simulink model "Maxom_fcs_noncascaded"  (R2025b)
settings: Solver=ode45  StartTime=0.0  StopTime=0.30  FixedStep=1e-6  MaxStep=1e-5  RelTol=1e-4  EnableMultiTasking=on
values from neighbouring files (symbols this model uses):
  Bfric = 0    [PMSMpara.m]
  ffai = 0.008667    [PMSMpara.m]
  Imax = 20    [PMSMpara.m]
  J = 0.044e-4    (= 4.4e-06)    [PMSMpara.m]
  kis = 0    [PMSMpara.m]
  kps = fsc*6.28*J/Kt    (= 0.364364007978)    [PMSMpara.m]
  Kt = np*1.5*ffai    (= 0.0910035)    [PMSMpara.m]
  Ld = Ls    (= 0.00045)    [PMSMpara.m]
  Lq = Ls    (= 0.00045)    [PMSMpara.m]
  np = 7    [PMSMpara.m]
  Rs = 0.5    [PMSMpara.m]
  Tcur = 1/32000    (= 3.125e-05)    [PMSMpara.m]
  Tpwm = 1/32000    (= 3.125e-05)    [PMSMpara.m]
  Tspd = 1/32000    (= 3.125e-05)    [PMSMpara.m]
  wn = 311040    [PMSMpara.m]
  zeta = 1    [PMSMpara.m]
undefined symbols (not defined in the file or in its folder): dspblkCoreblockFVToolHelper, gcbh
libraries: simulink x4, slpidlib x2, spsUniversalBridgeLib x1, spsCurrentMeasurementLib x1, EasyGo_Machine_lib x1, spsPermanentMagnetSynchronousMachineLib x1, spsSVPWMGenerator2LevelLib x1, spsDCVoltageSourceLib x1, sps_lib x1
(part 3 of 4)

== matlab function Maxom_fcs_noncascaded/f_pmsm_foc_sl/MATLAB Function12 ==
  data: ia input; gg output; ib input; ic input; id_ref input; we_ref input; we input; TL_hat input; theta_m input; Vdc input; Ld input; Lq input; Rs input; lambda_f input; Jm input; Bfric input; Tcur input; lambda_w input; lambda_id input; lambda_sw input; we_scale input; i_scale input; iq_max input; i_pred output; we_pred output; we_spread output
function [gg, i_pred, we_pred, we_spread] = fcs_noncascade_np3( ...
    ia, ib, ic, id_ref, we_ref, we, TL_hat, theta_m, ...
    Vdc, Ld, Lq, Rs, lambda_f, Jm, Bfric, Tcur, lambda_w,...
    lambda_id, lambda_sw, we_scale, i_scale, iq_max)
%#codegen
% Non-cascade FCS-MPC, Np=3, full 8^3 enumeration, normalized cost.
% NOMINAL model (electrical SMDO removed): current recursion keeps -Rs*i,
% no lumped current-disturbance compensation. TL_hat still feed-forwards load.

np = single(7);
ia=single(ia); ib=single(ib); ic=single(ic);
id_ref=single(id_ref); we_ref=single(we_ref); we=single(we); TL_hat=single(TL_hat);
Vdc=single(Vdc); Ld=single(Ld); Lq=single(Lq); Rs=single(Rs); lambda_f=single(lambda_f);
Jm=single(Jm); Bfric=single(Bfric); Ts=single(Tcur);
lambda_id=single(lambda_id); lambda_sw=single(lambda_sw);
we_scale=single(we_scale); i_scale=single(i_scale); iq_max=single(iq_max);

theta_e = single(mod(np*theta_m - pi/2, 2*pi));
inv_Ld=single(1)/Ld; inv_Lq=single(1)/Lq; inv_J=single(1)/Jm;
TsLd=Ts*inv_Ld; TsLq=Ts*inv_Lq;
ct=single(cos(theta_e)); st=single(sin(theta_e));

% --- hoisted constants ---
Kt     = single(1.5)*np*lambda_f;
aRd    = single(1) - TsLd*Rs;
aRq    = single(1) - TsLq*Rs;
TsKJ   = Ts*np*inv_J;
aW     = single(1) - Ts*Bfric*inv_J;
inv_ws=single(1)/we_scale; inv_is=single(1)/i_scale;
imax2 = iq_max*iq_max;
BIGPEN=single(1e5);
lsw3  = lambda_sw/single(3);

% Clarke/Park (measured)
i_alpha=(single(2)/3)*(ia-single(0.5)*ib-single(0.5)*ic);
i_beta =(single(2)/3)*(single(sqrt(3))/2)*(ib-ic);
is_d= ct*i_alpha+st*i_beta;
is_q=-st*i_alpha+ct*i_beta;

V=single([0 0 0;1 0 0;1 1 0;0 1 0;0 1 1;0 0 1;1 0 1;1 1 1]);
Kcl=(single(2)/3)*Vdc*single([1 -0.5 -0.5;0 single(sqrt(3))/2 -single(sqrt(3))/2]);

persistent s_prev
if isempty(s_prev)
    s_prev=zeros(3,1,'single');
end

% ===== nominal model: no disturbance bias =====
bd = single(0);   % was Ts*d_hat_d from SMDO
bq = single(0);   % was Ts*d_hat_q from SMDO

% ===== 8 dq voltages, and per-vector current INCREMENTS =====
Vab=Kcl*V';
Vdq=single([ct st;-st ct])*Vab;      % 2x8
dVd = TsLd*Vdq(1,:);                  % 1x8
dVq = TsLq*Vdq(2,:);

% ===== 8x8 switching table + sw0 from s_prev =====
SW = zeros(8,8,'single');
for a=1:8
    for b=1:8
        SW(a,b)=abs(V(b,1)-V(a,1))+abs(V(b,2)-V(a,2))+abs(V(b,3)-V(a,3));
    end
end
sw0=zeros(8,1,'single');
for n=1:8
    sw0(n)=abs(V(n,1)-s_prev(1))+abs(V(n,2)-s_prev(2))+abs(V(n,3)-s_prev(3));
end

% ===== horizon-3 tree search =====
g_best=single(1e30); n1_best=int32(1);
id_best=single(0); iq_best=single(0); we_best1=single(0);
we_min1=single(1e30); we_max1=single(-1e30);

for n1=1:8
    id1 = aRd*is_d + dVd(n1);
    iq1 = aRq*is_q + bq + dVq(n1);
    Te1 = Kt*iq1;
    we1 = aW*we + TsKJ*(Te1 - TL_hat);
    if we1<we_min1, we_min1=we1; end
    if we1>we_max1, we_max1=we1; end
    ew=(we_ref-we1)*inv_ws;
    ei=(id_ref-id1)*inv_is;
    c1 = ew*ew + lambda_id*(ei*ei) + lsw3*sw0(n1);
    if (id1*id1+iq1*iq1)>imax2, c1=c1+BIGPEN; end

    for n2=1:8
        id2 = aRd*id1 + bd + dVd(n2);
        iq2 = aRq*iq1 + bq + dVq(n2);
        Te2 = Kt*iq2;
        we2 = aW*we1 + TsKJ*(Te2 - TL_hat);
        ew=(we_ref-we2)*inv_ws; ei=(id_ref-id2)*inv_is;
        c12 = c1 + ew*ew + lambda_id*(ei*ei) + lsw3*SW(n1,n2);
        if (id2*id2+iq2*iq2)>imax2, c12=c12+BIGPEN; end

        for n3=1:8
            id3 = aRd*id2 + bd + dVd(n3);
            iq3 = aRq*iq2 + bq + dVq(n3);
            Te3 = Kt*iq3;
            we3 = aW*we2 + TsKJ*(Te3 - TL_hat);
            ew=(we_ref-we3)*inv_ws;
            ei=(id_ref-id3)*inv_is;
            Jc = c12 + lambda_w*(ew*ew) + lambda_id*(ei*ei) + lsw3*SW(n2,n3);
            if (id3*id3+iq3*iq3)>imax2, Jc=Jc+BIGPEN; end

            if Jc<g_best
                g_best=Jc; n1_best=int32(n1);
                id_best=id1; iq_best=iq1; we_best1=we1;
            end
        end
    end
end

s_prev=V(n1_best,:)';
Sa=s_prev(1); Sb=s_prev(2); Sc=s_prev(3);
gg=single([Sa;1-Sa;Sb;1-Sb;Sc;1-Sc]);
i_pred=single([id_best;iq_best]);
we_pred=single(we_best1);
we_spread=single(we_max1-we_min1);
end

== matlab function Maxom_fcs_noncascaded/f_pmsm_foc_sl/MATLAB Function13 ==
  data: ia input; gg output; ib input; ic input; id_ref input; we_ref input; we input; TL_hat input; theta_m input; Vdc input; Ld input; Lq input; Rs input; lambda_f input; Jm input; Bfric input; Tcur input; lambda_w input; lambda_id input; lambda_sw input; we_scale input; i_scale input; iq_max input
function gg = fcs_noncascade_np3_fast( ...
    ia, ib, ic, id_ref, we_ref, we, TL_hat, theta_m, ...
    Vdc, Ld, Lq, Rs, lambda_f, Jm, Bfric, Tcur, lambda_w, ...
    lambda_id, lambda_sw, we_scale, i_scale, iq_max)
%#codegen
%GPT optimized, 70 microseconds

% Optimized non-cascade FCS-MPC, Np = 3.
%
% Full 8^3 search is retained.
%
% Branch-and-bound assumes:
% lambda_w >= 0, lambda_id >= 0, lambda_sw >= 0.

%% Type conversion
ia        = single(ia);
ib        = single(ib);
ic        = single(ic);
id_ref    = single(id_ref);
we_ref    = single(we_ref);
we        = single(we);
TL_hat    = single(TL_hat);
theta_m   = single(theta_m);

Vdc       = single(Vdc);
Ld        = single(Ld);
Lq        = single(Lq);
Rs        = single(Rs);
lambda_f  = single(lambda_f);
Jm        = single(Jm);
Bfric     = single(Bfric);
Ts        = single(Tcur);

lambda_w  = single(lambda_w);
lambda_id = single(lambda_id);
lambda_sw = single(lambda_sw);
we_scale  = single(we_scale);
i_scale   = single(i_scale);
iq_max    = single(iq_max);

one = single(1);
np  = single(7);

%% Persistent constant lookup tables
persistent S SW alpha_pu beta_pu previous_index

if isempty(previous_index)

    % Switching-state order:
    % 1:000  2:100  3:110  4:010
    % 5:011  6:001  7:101  8:111
    S = single([ ...
        0 0 0;
        1 0 0;
        1 1 0;
        0 1 0;
        0 1 1;
        0 0 1;
        1 0 1;
        1 1 1]);

    % Hamming distance between switching states
    SW = single([ ...
        0 1 2 1 2 1 2 3;
        1 0 1 2 3 2 1 2;
        2 1 0 1 2 3 2 1;
        1 2 1 0 1 2 3 2;
        2 3 2 1 0 1 2 1;
        1 2 3 2 1 0 1 2;
        2 1 2 3 2 1 0 1;
        3 2 1 2 1 2 1 0]);

    % Normalized inverter voltage vectors:
    % v_alpha = Vdc*alpha_pu
    % v_beta  = Vdc*beta_pu
    alpha_pu = single([ ...
         0, ...
         0.6666666667, ...
         0.3333333333, ...
        -0.3333333333, ...
        -0.6666666667, ...
        -0.3333333333, ...
         0.3333333333, ...
         0]);

    beta_pu = single([ ...
         0, ...
         0, ...
         0.5773502692, ...
         0.5773502692, ...
         0, ...
        -0.5773502692, ...
        -0.5773502692, ...
         0]);

    % Initial switching state is 000
    previous_index = int32(1);
end

%% Electrical angle
theta_e = mod( ...
    np*theta_m - single(pi/2), ...
    single(2*pi));

ct = cos(theta_e);
st = sin(theta_e);

%% Clarke-Park transformation
two_thirds = single(0.6666666667);
half       = single(0.5);
sqrt3_half = single(0.8660254038);

i_alpha = two_thirds*(ia - half*ib - half*ic);
i_beta  = two_thirds*sqrt3_half*(ib - ic);

is_d =  ct*i_alpha + st*i_beta;
is_q = -st*i_alpha + ct*i_beta;

%% Hoisted model constants
TsLd = Ts/Ld;
TsLq = Ts/Lq;

aRd = one - TsLd*Rs;
aRq = one - TsLq*Rs;
aW  = one - Ts*Bfric/Jm;

Kt = single(1.5)*np*lambda_f;

% Original:
% we_next = aW*we + Ts*np/Jm*(Kt*iq - TL_hat)
%
% Combined form:
bIq = Ts*np*Kt/Jm;
dTL = Ts*np*TL_hat/Jm;

imax2 = iq_max*iq_max;

BIGPEN = single(1e5);

% Cost coefficients
kw12 = one/(we_scale*we_scale);
kw3  = lambda_w*kw12;
kid  = lambda_id/(i_scale*i_scale);
ksw  = lambda_sw/single(3);

%% dq voltage increments
kVd = TsLd*Vdc;
kVq = TsLq*Vdc;

dVd = zeros(1,8,'single');
dVq = zeros(1,8,'single');

for n = 1:8
    vd_pu =  ct*alpha_pu(n) + st*beta_pu(n);
    vq_pu = -st*alpha_pu(n) + ct*beta_pu(n);

    dVd(n) = kVd*vd_pu;
    dVq(n) = kVq*vq_pu;
end

%% Initial upper bound: repeat the previous state three times
p = previous_index;

id1 = aRd*is_d + dVd(p);
iq1 = aRq*is_q + dVq(p);
we1 = aW*we + bIq*iq1 - dTL;

ew = we_ref - we1;
ei = id_ref - id1;

g_best = kw12*ew*ew + kid*ei*ei;

if id1*id1 + iq1*iq1 > imax2
    g_best = g_best + BIGPEN;
end

id2 = aRd*id1 + dVd(p);
iq2 = aRq*iq1 + dVq(p);
we2 = aW*we1 + bIq*iq2 - dTL;

ew = we_ref - we2;
ei = id_ref - id2;

g_best = g_best + kw12*ew*ew + kid*ei*ei;

if id2*id2 + iq2*iq2 > imax2
    g_best = g_best + BIGPEN;
end

id3 = aRd*id2 + dVd(p);
iq3 = aRq*iq2 + dVq(p);
we3 = aW*we2 + bIq*iq3 - dTL;

ew = we_ref - we3;
ei = id_ref - id3;

g_best = g_best + kw3*ew*ew + kid*ei*ei;

if id3*id3 + iq3*iq3 > imax2
    g_best = g_best + BIGPEN;
end

n1_best = previous_index;

%% Horizon-three branch-and-bound search
for n1 = 1:8

    id1 = aRd*is_d + dVd(n1);
    iq1 = aRq*is_q + dVq(n1);
    we1 = aW*we + bIq*iq1 - dTL;

    ew = we_ref - we1;
    ei = id_ref - id1;

    c1 = kw12*ew*ew + kid*ei*ei ...
       + ksw*SW(previous_index,n1);

    if id1*id1 + iq1*iq1 > imax2
        c1 = c1 + BIGPEN;
    end

    % All remaining terms are nonnegative
    if c1 >= g_best
        continue;
    end

    for n2 = 1:8

        id2 = aRd*id1 + dVd(n2);
        iq2 = aRq*iq1 + dVq(n2);
        we2 = aW*we1 + bIq*iq2 - dTL;

        ew = we_ref - we2;
        ei = id_ref - id2;

        c12 = c1 ...
            + kw12*ew*ew ...
            + kid*ei*ei ...
            + ksw*SW(n1,n2);

        if id2*id2 + iq2*iq2 > imax2
            c12 = c12 + BIGPEN;
        end

        if c12 >= g_best
            continue;
        end

        for n3 = 1:8

            id3 = aRd*id2 + dVd(n3);
            iq3 = aRq*iq2 + dVq(n3);
            we3 = aW*we2 + bIq*iq3 - dTL;

            ew = we_ref - we3;
            ei = id_ref - id3;

            Jc = c12 ...
               + kw3*ew*ew ...
               + kid*ei*ei ...
               + ksw*SW(n2,n3);

            if id3*id3 + iq3*iq3 > imax2
                Jc = Jc + BIGPEN;
            end

            if Jc < g_best
                g_best  = Jc;
                n1_best = int32(n1);
            end
        end
    end
end

%% Apply first optimal switching state
previous_index = n1_best;

Sa = S(n1_best,1);
Sb = S(n1_best,2);
Sc = S(n1_best,3);

gg = [ ...
    Sa;
    one-Sa;
    Sb;
    one-Sb;
    Sc;
    one-Sc];

end

== matlab function Maxom_fcs_noncascaded/original ==
  data: ia input; gg output; ib input; ic input; id_ref input; iq_ref input; omega_mech input; theta_mech input; Vdc input; Ld input; Lq input; Rs input; lambda_f input; Tpwm input; lambda_w input; id1 output; id2 output; iq1 output; iq2 output
function [gg, id1, id2, iq1, iq2]  = fcs_mpc_2step(ia, ib, ic, id_ref, iq_ref, ...
                                      omega_mech, theta_mech, Vdc, ...
                                      Ld, Lq, Rs, lambda_f, Tpwm, lambda_w)
%#codegen
% =========================================================================
% TWO-STEP-DELAY FCS-MPC  --  compensating the one-sample compute delay
% -------------------------------------------------------------------------
% MEANING. On real hardware the vector chosen this tick cannot act during
%   [k,k+1): that interval was already committed last tick. So instead of
%   optimising from the measurement x(k), first roll the model forward one
%   step under the already-applied vector to get x(k+1), then choose the
%   vector for [k+1,k+2) by scoring the prediction x(k+2). The chosen vector
%   is stored and applied next cycle (via the actuation delay). This is the
%   classic Cortes et al. two-step scheme; horizon is otherwise 1.
% NEED. Without it, the controller assumes its choice takes effect
%   instantly. The real one-sample lag then shows up as extra current ripple
%   and, at high speed / high fundamental frequency, degraded stability --
%   the model and the plant are literally one step out of phase.
% WHEN TO USE. Any real deployment where prediction + optimisation consumes
%   a meaningful fraction of the tick (i.e. essentially always on an MCU),
%   or any simulation that models the actuation with a unit delay (z^-1) on
%   the output. In an idealised, instantaneous-actuation simulation it is
%   unnecessary. The same "predict one step first" idea composes with the
%   long-horizon and observer variants.
% =========================================================================

omega_r = omega_mech*7;
theta_e = mod(theta_mech*7-pi/2, 2*pi);

Ts = Tpwm;

% eight 2-level VSI switching states {Sa,Sb,Sc}
i_alpha = (2/3)*(ia - 0.5*ib - 0.5*ic);
i_beta = (2/3)*(sqrt(3)/2*(ib - ic));

% Park (align d with rotor flux)
is_d =  cos(theta_e)*i_alpha + sin(theta_e)*i_beta;
is_q = -sin(theta_e)*i_alpha + cos(theta_e)*i_beta;

V = single([0 0 0; 1 0 0; 1 1 0; 0 1 0; 0 1 1; 0 0 1; 1 0 1; 1 1 1]);
Kcl = (2/3)*Vdc*single([1 -0.5 -0.5; 0 sqrt(3)/2 -sqrt(3)/2]);

persistent s_now % vector applied during [k,k+1)
if isempty(s_now), s_now = zeros(3,1,'single'); end

% step 1: predict x(k+1) under the already-committed vector
Pk  = single([cos(theta_e) sin(theta_e); -sin(theta_e) cos(theta_e)]);
v0  = Pk * (Kcl * s_now);
id1 = is_d + Ts/Ld*(-Rs*is_d + omega_r*Lq*is_q + v0(1));
iq1 = is_q + Ts/Lq*(-Rs*is_q - omega_r*Ld*is_d - omega_r*lambda_f + v0(2));

% step 2: choose the vector for [k+1,k+2) at the advanced angle
th1 = theta_e + omega_r*Ts;
P1  = single([cos(th1) sin(th1); -sin(th1) cos(th1)]);
%P2  = single([cos(th2) sin(th2); -sin(th2) cos(th2)]);
g_best = single(inf);  idx = int32(1);
id2 = single(0);  iq2 = single(0); % declare outside the loop
for n = 1:8
    v_dq = P1 * (Kcl * V(n,:)');
    id2c = id1 + Ts/Ld*(-Rs*id1 + omega_r*Lq*iq1 + v_dq(1));
    iq2c = iq1 + Ts/Lq*(-Rs*iq1 - omega_r*Ld*id1 - omega_r*lambda_f + v_dq(2));
    g = (id_ref - id2c)^2 + lambda_w*(iq_ref - iq2c)^2;
    if g < g_best
        g_best = g;  idx = int32(n);
        id2 = id2c;  iq2 = iq2c; % keep the CHOSEN prediction
    end
end

s_new = V(idx,:)';
s_now = s_new; % becomes the committed vector next tick
Sa = s_new(1);  Sb = s_new(2);  Sc = s_new(3);
gg = single([Sa; 1-Sa; Sb; 1-Sb; Sc; 1-Sc]);
end

== matlab function Maxom_fcs_noncascaded/MATLAB Function1 ==
  data: speed_ref_cmd input; iq_feedforward output
function iq_feedforward = fcn_speed_feedforward( speed_ref_cmd)
    % ----------------- 系统硬参数定义 -----------------
    FS = single(32000);               % 控制频率 32kHz
    DT = single(1)/ FS;            % 采样周期 31.25us
    POLE_PAIRS = single(7);           % 极对数
    MAX_CURRENT_LIMIT = single(20); % 最大限流 20A (用于限制最大加速度)

    % ----------------- 电机软参数定义 (需要实测/辨识) -----------------
    % 1. J_total: 电机转子+负载的总转动惯量 (单位: kg·m^2)
    J_total = single(0.044e-4*2);        % 【需根据实际系统调整】
    % 2. Kt: 电机转矩常数 (单位: N·m/A)。通常 Kt ≈ 反电动势常数 Ke
    Kt = single(0.091003);                % 【需根据电机规格书调整】

    % ----------------- 持久化状态变量 -----------------
    persistent prev_ramped_speed ramped_speed
    if isempty(ramped_speed)
        prev_ramped_speed = single(0);
        ramped_speed = single(0);
    end

    persistent prev_iq_ff
if isempty(prev_iq_ff)
    prev_iq_ff = single(0);
end


    % ========================================================
    % 【第一步：速度轨迹规划（生成平滑斜坡）】
    % ========================================================
    % 理论最大加速度限制：a_max = (Kt * Max_Current) / J_total
    max_accel_rpm_s = (Kt * MAX_CURRENT_LIMIT) / J_total * 60.0 / (2 * pi);

    % 跟随目标速度（做斜坡上升/下降限制）
    if speed_ref_cmd > ramped_speed
        ramped_speed = ramped_speed + max_accel_rpm_s * DT; % 加速
        if ramped_speed > speed_ref_cmd
            ramped_speed = speed_ref_cmd;
        end
    elseif speed_ref_cmd < ramped_speed
        ramped_speed = ramped_speed - max_accel_rpm_s * DT; % 减速
        if ramped_speed < speed_ref_cmd
            ramped_speed = speed_ref_cmd;
        end
    end

    % ========================================================
    % 【第二步：计算加速度前馈】
    % ========================================================
    % 1. 计算速度差分（得到实际需要的加速度）
    delta_rpm = ramped_speed - prev_ramped_speed;
    accel_rpm_s = delta_rpm / DT; % RPM / s

    % 2. 将加速度转换为 电角速度 变化率 (rad/s^2)
    accel_rad_s2 = accel_rpm_s * (2 * pi / 60.0) * POLE_PAIRS;

    % 3. 计算所需的前馈 Iq 电流 (基于牛顿第二定律: T = J * a, T = Kt * Iq)
    iq_raw = (J_total * accel_rad_s2) / Kt;

    % --- 引入前馈斜率限制（替代低通滤波，0相位滞后） ---

% 设定前馈电流的最大变化率（单位：A/s）
% 根据电机电气时间常数，建议从 500 ~ 2000 A/s 开始往下调
MAX_FF_SLEW_RATE = single(50000); 
max_delta_per_loop = MAX_FF_SLEW_RATE * DT; % 每个控制周期允许的最大电流变化

diff = iq_raw - prev_iq_ff;
if diff > max_delta_per_loop
    diff = max_delta_per_loop;
elseif diff < -max_delta_per_loop
    diff = -max_delta_per_loop;
end

% 得到平滑后的前馈（方波的垂直边变成了斜坡边）
iq_feedforward = prev_iq_ff + diff;

% 最后统一做安全限幅
iq_feedforward = max(-MAX_CURRENT_LIMIT, min(MAX_CURRENT_LIMIT, iq_feedforward));
prev_iq_ff = iq_feedforward;

    % 4. 安全限幅（防止前馈计算出超出硬件能力的电流）
    if iq_feedforward > MAX_CURRENT_LIMIT
        iq_feedforward = MAX_CURRENT_LIMIT;
    elseif iq_feedforward < -MAX_CURRENT_LIMIT
        iq_feedforward = -MAX_CURRENT_LIMIT;
    end

    % 更新状态
    prev_ramped_speed = ramped_speed;
end

== matlab function Maxom_fcs_noncascaded/MATLAB Function3 ==
  data: spd_ref input; iq_total output; spd_act input; iq_ff input
function iq_total = fcn_PI_FF_AntiWindup(spd_ref, spd_act, iq_ff)
    % ------------ 系统硬参数定义 ------------
    FS = single(32000);
    DT = single(1)/FS;  % 采样周期 31.25us
    Kp = single(1.5);   % 比例系数（请根据您原来 PID 的参数修改）
    Ki = single(50.0);  % 积分系数（请根据您原来 PID 的参数修改）
    
    MAX_LIM = single(20);    % 上限幅 (跟您外部的 20A 保持一致)
    MIN_LIM = single(-20);   % 下限幅
    
    persistent integral
    if isempty(integral)
        integral = single(0);
    end
    
    % 1. 计算速度误差
    error = spd_ref - spd_act;
    
    % 2. 计算 PI 输出 + 前馈 的总和
    iq_total_raw = (Kp * error + integral) + iq_ff;
    
    % 3. 对总和进行外部限幅
    if iq_total_raw > MAX_LIM
        iq_total = MAX_LIM;
    elseif iq_total_raw < MIN_LIM
        iq_total = MIN_LIM;
    else
        iq_total = iq_total_raw;
    end
    
    % 4. 【核心】：感知外部限幅的真实抗饱和策略
    % 如果触发了限幅，且误差方向还试图让限幅更深，则冻结积分器！
    if (iq_total >= MAX_LIM && error > 0) || (iq_total <= MIN_LIM && error < 0)
        integral = integral; % 冻结积分
    else
        integral = integral + Ki * error * DT; % 正常累加积分
    end
end

== matlab function Maxom_fcs_noncascaded/f_pmsm_foc_sl/MATLAB Function7 ==
  data: ia input; gg output; ib input; ic input; id_ref input; iq_ref input; omega_mech input; theta_mech input; Vdc input; Ld input; Lq input; Rs input; lambda_f input; Tcur input; lambda_w input; Va output; Vb output; Vc output
function [gg, Va, Vb, Vc] = fcs_smdo_2step(ia, ib, ic, id_ref, iq_ref, ...
                                     omega_mech, theta_mech, Vdc, Ld, Lq, Rs, ...
                                     lambda_f, Tcur, lambda_w)
%#codegen
% ---- horizon & dims (INTEGERS — do not make these single) --------------
Np   = int32(3);            % prediction horizon
dim  = int32(3 * Np);
ny   = int32(2);
nyNp = int32(ny * Np);

% ---- pole pairs & electrical quantities (separate from horizon) --------
omega_r  = single(omega_mech*7);               % electrical if external np gain applied;
theta_e = mod(theta_mech*7 - pi/2, 2*pi);
Ts = single(Tcur);

% Clarke + Park
i_alpha = (2/3)*(ia - 0.5*ib - 0.5*ic);
i_beta  = (2/3)*(sqrt(3)/2*(ib - ic));
is_d =  cos(theta_e)*i_alpha + sin(theta_e)*i_beta;
is_q = -sin(theta_e)*i_alpha + cos(theta_e)*i_beta;


% ---- constants that were input ports in v2 -----------------------------
lambda_u = single(1e-3);     % switching-effort weight; 0 = pure tracking to start
en_pwm   = true;            % no FSM gate yet -> always enabled
en_tsc   = false;           % INSTANTANEOUS actuation in this sim -> TSC OFF

KB  = int32(4);          % K-best width  (Kb). 62 node evals at Np=3.
NC  = int32(2 * KB);     % candidate buffer width

% SMDO gains (Sun 2020, Eq. 17, l = 2)
% alpha_i = i*ab - (i-1), beta_i = i*bb - (i-1), ab in (1-i1,1), bb in (1,1+i2)
OBS_AB = single(0.8);  % alpha-bar -> alpha1=0.8, alpha2=0.6
OBS_BB = single(1.2); % beta-bar -> beta1 =1.2, beta2 =1.4
OBS_K1 = single(6000); % kappa1 = kappa2  (A1, A2 Hurwitz)
OBS_K2 = single(6000);
OBS_K3 = single(4e6); % kappa3 = kappa4
OBS_K4 = single(4e6);
% Forward-Euler discretisation verified stable at Ts = 31.25 us
% (kappa1*Ts = 0.19 << 1). Convergence ~ 5-10 ms in closed loop.

U_SET = single([0; 1]);

is_d     = single(is_d);      is_q     = single(is_q);
id_ref   = single(id_ref);    iq_ref   = single(iq_ref);
omega_r  = single(omega_r);   theta_e  = single(theta_e);
Vdc      = single(Vdc);       Ld       = single(Ld);
Lq       = single(Lq);        Rs       = single(Rs);
lambda_f = single(lambda_f);  Ts       = single(Ts);
lambda_u = single(lambda_u);  lambda_w = single(lambda_w);

if ~en_pwm
    Va = single(0); Vb = single(0); Vc = single(0);
    return;
end

% s_apply_now: vector applied during the UPCOMING interval [k, k+1)
% s_applied: vector applied during the ELAPSED interval [k-1, k)
persistent s_apply_now s_applied U_opt_prev z1 z2
if isempty(s_apply_now)
    s_apply_now = zeros(3, 1, 'single');
    s_applied   = zeros(3, 1, 'single');
    U_opt_prev  = zeros(dim, 1, 'single');
    z1 = single([is_d; is_q]);  % observer state estimate
    z2 = zeros(2, 1, 'single'); % lumped disturbance estimate [A/s]
end

x_k = single([is_d; is_q]);

% [U2] SMDO UPDATE  (Sun 2020, Eq. 17) 
% Uses the voltage that was ACTUALLY applied over the elapsed interval,
% reconstructed at the previous sample angle.
th_prev = theta_e - omega_r * Ts;
ctp = single(cos(th_prev));  stp = single(sin(th_prev));
K_cl_p = single((2/3) * Vdc * [1, -0.5, -0.5; 0, sqrt(3)/2, -sqrt(3)/2]);
v_dq_applied = single([ctp, stp; -stp, ctp]) * (K_cl_p * s_applied);

e_obs = z1 - x_k; % z1 - x
% sig(e,a) = |e|^a * sign(e)
sig_a1 = abs(e_obs).^OBS_AB          .* sign(e_obs); % alpha1 = ab
sig_b1 = abs(e_obs).^OBS_BB          .* sign(e_obs); % beta1  = bb
sig_a2 = abs(e_obs).^(2*OBS_AB - 1)  .* sign(e_obs); % alpha2 = 2ab-1
sig_b2 = abs(e_obs).^(2*OBS_BB - 1)  .* sign(e_obs); % beta2  = 2bb-1

f_nom = single([(-Rs*x_k(1) + omega_r*Lq*x_k(2)) / Ld; ...
                (-Rs*x_k(2) - omega_r*Ld*x_k(1) - omega_r*lambda_f) / Lq]);
g_u   = single([v_dq_applied(1)/Ld; v_dq_applied(2)/Lq]);

z1 = z1 + Ts * (f_nom + g_u + z2 - OBS_K1*sig_a1 - OBS_K2*sig_b1);
z2 = z2 + Ts * (          - OBS_K3*sig_a2 - OBS_K4*sig_b2);
d_hat = z2; % [A/s], per axis

%  DISCRETE MODEL WITH d_hat INJECTED 
A_mat = single([1 - Ts*Rs/Ld,        Ts*omega_r*Lq/Ld;
                -Ts*omega_r*Ld/Lq,   1 - Ts*Rs/Lq]);
d_vec = single([0; -Ts*omega_r*lambda_f/Lq]) + Ts * d_hat; % [U2] injection

% [U1] TSC: ADVANCE THE PREDICTION START 
if en_tsc
    % x(k+1) under the vector currently being applied, at angle theta_e
    ct0 = single(cos(theta_e));  st0 = single(sin(theta_e));
    B_sw0 = single([Ts/Ld, 0; 0, Ts/Lq]) * ...
            (single([ct0, st0; -st0, ct0]) * K_cl_p);
    x0  = A_mat * x_k + B_sw0 * s_apply_now + d_vec;
    th0 = theta_e + omega_r * Ts;% B_sw for the optimised interval 
    s_ref = s_apply_now; % switching-effort reference = u(k)
else
    x0  = x_k;
    th0 = theta_e;
    s_ref = s_apply_now;
end

ct = single(cos(th0));  st = single(sin(th0));
B_sw = single([Ts/Ld, 0; 0, Ts/Lq]) * ...
       (single([ct, st; -st, ct]) * K_cl_p);

%  BUILD PREDICTION MATRICES (as v1) 
AiB = zeros(ny, 3, Np, 'single');
temp_A = single(eye(ny));
for p = 1:Np
    AiB(:,:,p) = temp_A * B_sw;
    temp_A = temp_A * A_mat;
end

Upsilon = zeros(nyNp, dim, 'single');
Y_free  = zeros(nyNp, 1,   'single');
Y_star  = zeros(nyNp, 1,   'single');
A_j   = single(eye(ny));
sum_d = single(zeros(ny, 1));
for j = 1:Np
    sum_d = A_mat * sum_d + d_vec;
    A_j   = A_j * A_mat;
    r1 = ny*(j-1) + 1; 
    yk = A_j * x0 + sum_d;
    Y_free(r1) = yk(1);
    Y_free(r1+1)= yk(2);
    Y_star(r1) = id_ref;
    Y_star(r1+1) = iq_ref;
    for m = 1:j
        pw = j - m;
        blk = AiB(:, :, pw+1);
        cb = 3*(m-1);
        for rr = 1:ny
            for cc = 1:3
                Upsilon(r1+rr-1, cb+cc) = blk(rr, cc);
            
            
        end
    end 
        
    end
end

Smat = zeros(dim, dim, 'single');
Emat = zeros(dim, 3,   'single');
for p = 1:Np
    r1 = 3*(p-1) + 1;
    Smat(r1, r1) = single(1);
    Smat (r1+1, r1+1) = single(1);
    Smat(r1+2, r1+2) = single(1);
    if p > 1
        Smat(r1, r1-3) = single(-1);
        Smat(r1+1, r1-2) = single(-1);
        Smat(r1+2, r1-1) = single(-1);
    end
end
Emat(1:3, 1:3) = eye(3, 'single');

Q_tilde = zeros(nyNp, nyNp, 'single');
for p = 1:Np
    idx = ny*(p-1);
    Q_tilde(idx+1, idx+1) = single(1);
    Q_tilde(idx+2, idx+2) = lambda_w;
end

H = (Upsilon') * Q_tilde * Upsilon  +  lambda_u * (Smat' * Smat);
for p = 1:dim
    H(p,p) = H(p,p) + single(1e-8);
end

e_ref = Y_star - Y_free;
Theta = -(Upsilon' * (Q_tilde * e_ref)) - lambda_u * (Smat' * (Emat * s_ref));
S_unc = -(H \ Theta);
R = chol(H);                       % upper triangular, R'*R = H

% ================ [U3] K-BEST SPHERE DECODING (Zafra 2022) ===============
% Breadth-first over layers i = dim ... 1. At each layer every survivor is
% expanded with u in {0,1}; partial distance (Zafra Eq. 10):
%   d(i) = ( sum_{j=i..dim} R(i,j)*(S(j)-S_unc(j)) )^2 + d(i+1)
% Only the KB cheapest survive. Fixed node count:
%   sum_i min(2*nsurv, 2*KB)  = 62 evaluations for Np=3, KB=4.
surv  = zeros(dim, KB, 'single');   scost = zeros(1, KB, 'single');
cand  = zeros(dim, NC, 'single');   ccost = zeros(1, NC, 'single');
nsurv = int32(1);                   scost(1) = single(0);

for i = dim:-1:1
    ncand = int32(0);
    for s = 1:nsurv
        for c = 1:2
            ncand = ncand + int32(1);
            cand(:, ncand) = surv(:, s);
            cand(i, ncand) = U_SET(c);
            z = single(0);
            for j = i:dim
                z = z + R(i,j) * (cand(j, ncand) - S_unc(j));
            end
            ccost(ncand) = scost(s) + z*z;
        end
    end
    % partial selection sort: move the KB cheapest to the front
    nkeep = min(ncand, KB);
    for a = 1:nkeep
        bidx = a;
        for b = a+1:ncand
            if ccost(b) < ccost(bidx), bidx = b; end
        end
        if bidx ~= a
            tmpc = ccost(a); ccost(a) = ccost(bidx); ccost(bidx) = tmpc;
            tmpv = cand(:, a); cand(:, a) = cand(:, bidx); cand(:, bidx) = tmpv;
        end
    end
    for kk = 1:KB
        if kk <= nkeep
            surv(:, kk) = cand(:, kk);
            scost(kk) = ccost(kk);
        end
    end
    nsurv = nkeep;
end

% best survivor
bi = int32(1);
for s = 2:nsurv
    if scost(s) < scost(bi), bi = s; end
end
S_opt  = surv(:, bi);
c_best = scost(bi);

% warm-start guarantee: time-shifted previous optimum, take if cheaper
S_ws = zeros(dim, 1, 'single');
S_ws(1:dim-3)     = U_opt_prev(4:dim);
S_ws(dim-2:dim)   = U_opt_prev(dim-2:dim);
dws = R * (S_ws - S_unc);
c_ws = dws' * dws;
if c_ws < c_best
    S_opt = S_ws;
end

% ============================ OUTPUT & STATE =============================


Sa = S_opt(1);  Sb = S_opt(2);  Sc = S_opt(3);
Va = single((2*Sa - Sb - Sc) / 3) * Vdc;
Vb = single((2*Sb - Sa - Sc) / 3) * Vdc;
Vc = single((2*Sc - Sa - Sb) / 3) * Vdc;

U_opt_prev = S_opt;
if en_tsc
    % selected vector acts during [k+1, k+2); the vector acting during
    % [k, k+1) was decided last cycle -> it is the "elapsed" one next call.
    s_applied   = s_apply_now;
    s_apply_now = single([Sa; Sb; Sc]);
else
    % instantaneous actuation: selected vector acts during [k, k+1),
    % so it is also the elapsed-interval vector at the next call.
    s_apply_now = single([Sa; Sb; Sc]);
    s_applied   = s_apply_now;
end



% ---- output: gates for your 6-pulse bridge -----------------------------
% v2 already computed Sa,Sb,Sc = S_opt(1:3) inside the body.
gg = single([S_opt(1); 1-S_opt(1); ...
             S_opt(2); 1-S_opt(2); ...
             S_opt(3); 1-S_opt(3)]);



% Va,Vb,Vc still returned if you want to scope them, but the BRIDGE uses gg.
end

== matlab function Maxom_fcs_noncascaded/original3 ==
  data: ia input; gA output; gB output; d output; ib input; ic input; id_ref input; iq_ref input; omega_mech input; theta_mech input; Vdc input; Ld input; Lq input; Rs input; lambda_f input; Ts input; lambda_w input
function [gA, gB, d] = fcs_2vec(ia, ib, ic, id_ref, iq_ref, ...
                                omega_mech, theta_mech, Vdc, Ld, Lq, Rs, ...
                                lambda_f, Ts, lambda_w)
%#codegen
np = single(7);
we = single(omega_mech*np);
th = mod(theta_mech*np - pi/2, 2*pi);     

% Clarke + Park -> measured dq current
a = (2/3)*(ia - 0.5*ib - 0.5*ic);
b = (2/3)*(sqrt(3)/2*(ib - ic));
id =  cos(th)*a + sin(th)*b;
iq = -sin(th)*a + cos(th)*b;
i    = single([id; iq]);
iref = single([id_ref; iq_ref]);
W    = single([1 0; 0 lambda_w]);

% 6 active vectors (columns)
V = single([1 1 0 0 0 1; 0 1 1 1 0 0; 0 0 0 1 1 1]);

% slope common to all vectors (null-vector slope, vd=vq=0)
s0 = single([(-Rs*id + we*Lq*iq)/Ld; ...
             (-Rs*iq - we*Ld*id - we*lambda_f)/Lq]);

Kdq = single([cos(th) sin(th); -sin(th) cos(th)]);   % Park matrix

% --- select best active vector (full-period cost as the selector) ---
bestc  = single(1e30);
bi     = int32(1);
sa_best = s0;
for k = 1:6
    s = V(:,k);
    vabc = (Vdc/3)*single([2*s(1)-s(2)-s(3); ...
                           2*s(2)-s(1)-s(3); ...
                           2*s(3)-s(1)-s(2)]);
    va = (2/3)*(vabc(1) - 0.5*vabc(2) - 0.5*vabc(3));
    vb = (2/3)*(sqrt(3)/2*(vabc(2) - vabc(3)));
    vdq = Kdq*single([va; vb]);
    sa  = s0 + single([vdq(1)/Ld; vdq(2)/Lq]);   % slope under this vector
    e   = iref - (i + Ts*sa);                     % end-of-period error
    c   = e'*W*e;
    if c < bestc
        bestc = c; bi = int32(k); sa_best = sa;
    end
end

% --- optimal duty of active vs null (least-squares deadbeat) ---
Del = (iref - i)/Ts;
num = (Del - s0)'*W*(sa_best - s0);
den = (sa_best - s0)'*W*(sa_best - s0) + single(1e-9);
d   = min(max(num/den, single(0)), single(1));

% --- gate patterns ---
sA = V(:,bi);
gA = single([sA(1); 1-sA(1); sA(2); 1-sA(2); sA(3); 1-sA(3)]);  % active
gB = single([0; 1; 0; 1; 0; 1]);                                % null [0 0 0]
end

== matlab function Maxom_fcs_noncascaded/f_pmsm_foc_sl/original1 ==
  data: ia input; gA output; gB output; d output; ib input; ic input; id_ref input; iq_ref input; omega_mech input; theta_mech input; Vdc input; Ld input; Lq input; Rs input; lambda_f input; Tpwm input; lambda_w input
function [gA, gB, d] = fcs_2vec(ia, ib, ic, id_ref, iq_ref, ...
                                omega_mech, theta_mech, Vdc, Ld, Lq, Rs, ...
                                lambda_f, Tpwm, lambda_w)
%#codegen
np = single(7);
we = single(omega_mech*np);
th = mod(theta_mech*np - pi/2, 2*pi); 
Ts = Tpwm/2;

% Clarke + Park -> measured dq current
a = (2/3)*(ia - 0.5*ib - 0.5*ic);
b = (2/3)*(sqrt(3)/2*(ib - ic));
id =  cos(th)*a + sin(th)*b;
iq = -sin(th)*a + cos(th)*b;
i    = single([id; iq]);
iref = single([id_ref; iq_ref]);
W    = single([1 0; 0 lambda_w]);



% 6 active vectors (columns)
V = single([1 1 0 0 0 1; 0 1 1 1 0 0; 0 0 0 1 1 1]);

% slope common to all vectors (null-vector slope, vd=vq=0)
s0 = single([(-Rs*id + we*Lq*iq)/Ld; ...
             (-Rs*iq - we*Ld*id - we*lambda_f)/Lq]);

Kdq = single([cos(th) sin(th); -sin(th) cos(th)]);   % Park matrix

% --- select best active vector (full-period cost as the selector) ---
bestc  = single(1e30);
bi     = int32(1);
sa_best = s0;
for k = 1:6
    s = V(:,k);
    vabc = (Vdc/3)*single([2*s(1)-s(2)-s(3); ...
                           2*s(2)-s(1)-s(3); ...
                           2*s(3)-s(1)-s(2)]);
    va = (2/3)*(vabc(1) - 0.5*vabc(2) - 0.5*vabc(3));
    vb = (2/3)*(sqrt(3)/2*(vabc(2) - vabc(3)));
    vdq = Kdq*single([va; vb]);
    sa  = s0 + single([vdq(1)/Ld; vdq(2)/Lq]);   % slope under this vector
    e   = iref - (i + Ts*sa);                     % end-of-period error
    c   = e'*W*e;
    if c < bestc
        bestc = c; bi = int32(k); sa_best = sa;
    end
end

% --- optimal duty of active vs null (least-squares deadbeat) ---
Del = (iref - i)/Ts;
num = (Del - s0)'*W*(sa_best - s0);
den = (sa_best - s0)'*W*(sa_best - s0) + single(1e-9);
d   = min(max(num/den, single(0)), single(1));

% --- gate patterns ---
sA = V(:,bi);
gA = single([sA(1); 1-sA(1); sA(2); 1-sA(2); sA(3); 1-sA(3)]);  % active
gB = single([0; 1; 0; 1; 0; 1]);                                % null [0 0 0]
end

== matlab function Maxom_fcs_noncascaded/ang_comp2 ==
  data: real_ang input; real_ang_pu output
function real_ang_pu = fcn(real_ang)
%#codegen

while(real_ang > 1)
    real_ang = real_ang - single(1);
end

while(real_ang < 0)
    real_ang = real_ang + single(1);
end

real_ang_pu = real_ang;

== matlab function Maxom_fcs_noncascaded/original2 ==
  data: ia input; gg output; ib input; ic input; id_ref input; iq_ref input; omega_mech input; theta_mech input; Vdc input; Ld input; Lq input; Rs input; lambda_f input; Tcur input; lambda_w input; id1 output; id2 output; iq1 output; iq2 output; v_ab_out output
function [gg, id1, id2, iq1, iq2, v_ab_out] = fcs_mpc_3step(ia, ib, ic, id_ref, iq_ref, ...
                                      omega_mech, theta_mech, Vdc, ...
                                      Ld, Lq, Rs, lambda_f, Tcur, lambda_w)
%#codegen
% =========================================================================
% DELAY-COMPENSATED FCS-MPC, PREDICTION HORIZON N = 3
%   1) roll x(k) -> x(k+1) under the already-committed vector (delay comp)
%   2) search all 8^3 vector SEQUENCES over [k+1,k+4), sum the stage cost
%   3) apply only the FIRST vector of the best sequence, store it, recede
%   Greedy per-step selection is NOT equivalent -- the sequence search is
%   what makes this a true horizon-3 controller.
% =========================================================================
omega_r = omega_mech*7;
theta_e = mod(theta_mech*7, 2*pi);

Ts = Tcur/2;

% measured currents -> dq
i_alpha = (2/3)*(ia - 0.5*ib - 0.5*ic);
i_beta  = (2/3)*(sqrt(3)/2*(ib - ic));
is_d =  cos(theta_e)*i_alpha + sin(theta_e)*i_beta;
is_q = -sin(theta_e)*i_alpha + cos(theta_e)*i_beta;

V   = single([0 0 0; 1 0 0; 1 1 0; 0 1 0; 0 1 1; 0 0 1; 1 0 1; 1 1 1]);
Kcl = (2/3)*Vdc*single([1 -0.5 -0.5; 0 sqrt(3)/2 -sqrt(3)/2]);
Vab = Kcl * V.';                         % 2x8 alpha-beta voltage per vector

persistent s_now                         % vector applied during [k,k+1)
if isempty(s_now), s_now = zeros(3,1,'single'); end

% --- step 1: delay compensation, x(k) -> x(k+1) under committed vector ----
Pk  = single([cos(theta_e) sin(theta_e); -sin(theta_e) cos(theta_e)]);
v0  = Pk * (Kcl * s_now);
id1 = is_d + Ts/Ld*(-Rs*is_d + omega_r*Lq*is_q + v0(1));
iq1 = is_q + Ts/Lq*(-Rs*is_q - omega_r*Ld*is_d - omega_r*lambda_f + v0(2));

% --- per-step dq voltages of all 8 vectors at the 3 horizon angles --------
th1 = theta_e + omega_r*Ts;
th2 = theta_e + 2*omega_r*Ts;
th3 = theta_e + 3*omega_r*Ts;
Vdq1 = single([cos(th1) sin(th1); -sin(th1) cos(th1)]) * Vab;
Vdq2 = single([cos(th2) sin(th2); -sin(th2) cos(th2)]) * Vab;
Vdq3 = single([cos(th3) sin(th3); -sin(th3) cos(th3)]) * Vab;

% --- step 2: search all 8^3 sequences, sum stage cost --------------------
g_best   = single(inf);
idx1     = int32(1);
id2_best = single(0);  iq2_best = single(0);
for a = 1:8
    [ida, iqa] = predict(id1, iq1, Vdq1(1,a), Vdq1(2,a), Ts, Ld, Lq, Rs, omega_r, lambda_f);
    ga = (id_ref - ida)^2 + lambda_w*(iq_ref - iqa)^2;         % stage cost k+2
    for b = 1:8
        [idb, iqb] = predict(ida, iqa, Vdq2(1,b), Vdq2(2,b), Ts, Ld, Lq, Rs, omega_r, lambda_f);
        gb = (id_ref - idb)^2 + lambda_w*(iq_ref - iqb)^2;     % stage cost k+3
        for c = 1:8
            [idc, iqc] = predict(idb, iqb, Vdq3(1,c), Vdq3(2,c), Ts, Ld, Lq, Rs, omega_r, lambda_f);
            gc = (id_ref - idc)^2 + lambda_w*(iq_ref - iqc)^2; % stage cost k+4
            J = ga + gb + gc;
            if J < g_best
                g_best   = J;
                idx1     = int32(a);        % FIRST vector of the best sequence
                id2_best = ida;  iq2_best = iqa;
            end
        end
    end
end

% --- apply first vector, store for next tick's delay comp ----------------
s_now = V(idx1,:).';
Sa = s_now(1);  Sb = s_now(2);  Sc = s_now(3);
gg  = [Sa; ~Sa; Sb; ~Sb; Sc; ~Sc];

id2 = id2_best;   iq2 = iq2_best; % predicted x(k+2) of chosen 1st vector
v_ab_out = Vab(:, idx1);                    % alpha-beta voltage of applied vector
end

% -------------------------------------------------------------------------
function [idn, iqn] = predict(id, iq, vd, vq, Ts, Ld, Lq, Rs, wr, lf)
    idn = id + Ts/Ld*(-Rs*id + wr*Lq*iq + vd);
    iqn = iq + Ts/Lq*(-Rs*iq - wr*Ld*id - wr*lf + vq);
end

== matlab function Maxom_fcs_noncascaded/f_pmsm_foc_sl/MATLAB Function5 ==
  data: ia input; gg output; ib input; ic input; id_ref input; iq_ref input; omega_mech input; theta_mech input; Vdc input; Ld input; Lq input; Rs input; lambda_f input; Tcur input; lambda_w input
function gg  = fcs_smdo_1step(ia, ib, ic, id_ref, iq_ref, ...
                                     omega_mech, theta_mech, Vdc, Ld, Lq, Rs, ...
                                     lambda_f, Tcur, lambda_w)
%#codegen
omega_r = single(omega_mech);
theta_e = single(mod(theta_mech * 7 - pi/2, 2*pi));
Ts      = single(Tcur);

Vdc = single(Vdc);  Ld = single(Ld);  Lq = single(Lq);  Rs = single(Rs);
lambda_f = single(lambda_f);  lambda_w = single(lambda_w);
id_ref   = single(id_ref);    iq_ref   = single(iq_ref);

% precompute reciprocals: divides are ~14 cycles on M4/M7, multiplies ~1
inv_Ld = single(1)/Ld;
inv_Lq = single(1)/Lq;
TsLd   = Ts*inv_Ld;
TsLq   = Ts*inv_Lq;

ct = single(cos(theta_e));  st = single(sin(theta_e));

i_alpha = (2/3)*(ia - 0.5*ib - 0.5*ic);
i_beta  = (2/3)*(sqrt(3)/2*(ib - ic));
is_d = single( ct*i_alpha + st*i_beta);
is_q = single(-st*i_alpha + ct*i_beta);
x_k  = single([is_d; is_q]);

AB = single(0.6);  BB = single(1.2);
K1 = single(6000); K2 = single(6000);
K3 = single(2.5e5); K4 = single(1e6);

V   = single([0 0 0; 1 0 0; 1 1 0; 0 1 0; 0 1 1; 0 0 1; 1 0 1; 1 1 1]);
Kcl = (2/3)*Vdc*single([1 -0.5 -0.5; 0 sqrt(3)/2 -sqrt(3)/2]);

persistent z1 z2 s_prev
if isempty(z1)
    z1     = x_k;
    z2     = zeros(2,1,'single');
    s_prev = zeros(3,1,'single');
end

% ===================== SMDO UPDATE =====================
th_p = theta_e - omega_r*Ts;
ctp  = single(cos(th_p));  stp = single(sin(th_p));
v_app = single([ctp stp; -stp ctp]) * (Kcl * s_prev);

e = z1 - x_k;
ae = abs(e);  se = sign(e);
sa1 = ae.^AB        .* se;   sb1 = ae.^BB        .* se;
sa2 = ae.^(2*AB-1)  .* se;   sb2 = ae.^(2*BB-1)  .* se;

f_nom = single([(-Rs*x_k(1) + omega_r*Lq*x_k(2)) * inv_Ld; ...
                (-Rs*x_k(2) - omega_r*Ld*x_k(1) - omega_r*lambda_f) *inv_Lq]);
g_u   = single([v_app(1)*inv_Ld; v_app(2)*inv_Lq]);

z1 = z1 + Ts*(f_nom + g_u + z2 - K1*sa1 - K2*sb1);
z2 = z2 + Ts*(- K3*sa2 - K4*sb2);
d_hat = z2;

% ===================== PRECOMPUTE 8 dq VOLTAGES (once) =====================
% Vdq(:,n) = P0 * (Kcl * V(n,:)') for all 8 states, built without the loop.
% Kcl*V' gives the 8 alpha-beta vectors; P0 rotates them into dq.
Vab = Kcl * V';                          % 2x8, all alpha-beta voltages
Vdq = single([ct st; -st ct]) * Vab;     % 2x8, all dq voltages (P0 applied once)

% ===================== CONSTANT PART OF PREDICTION (once) =================
% These don't depend on n -- pulling them out of the loop is the main win.

id_base = is_d + TsLd*(-Rs*is_d + omega_r*Lq*is_q)                    + Ts*d_hat(1);
iq_base = is_q + TsLq*(-Rs*is_q - omega_r*Ld*is_d - omega_r*lambda_f) + Ts*d_hat(2);

% ===================== SINGLE-STEP SEARCH =====================
g_best = single(9e20);  idx = int32(1);
for n = 1:8
    id_p = id_base + TsLd*Vdq(1,n);      % only the vector-dependent term remains
    iq_p = iq_base + TsLq*Vdq(2,n);
    ed = id_ref - id_p;
    eq = iq_ref - iq_p;
    g  = ed*ed + lambda_w*(eq*eq);
    if g < g_best
        g_best = g;  idx = int32(n);
    end
end

s_new  = V(idx,:)';
s_prev = s_new;
Sa = s_prev(1);  Sb = s_prev(2);  Sc = s_prev(3);

gg = single([Sa; 1-Sa; Sb; 1-Sb; Sc; 1-Sc]);

end

== matlab function Maxom_fcs_noncascaded/f_pmsm_foc_sl/MATLAB Function6 ==
  data: theta_e input; we_raw output; Ts input
function we_raw = speed_deriv(theta_e, Ts)
%#codegen
% theta_e is PER-UNIT: 1.0 = one full electrical revolution
persistent th_prev
if isempty(th_prev), th_prev = theta_e; end
de = theta_e - th_prev;
if de >  0.5,  de = de - 1;      % wrap is ±1 in per-unit, not ±2*pi
elseif de < -0.5, de = de + 1;
end
we_raw = de / Ts;                % electrical rev/s
th_prev = theta_e;
end

== matlab function Maxom_fcs_noncascaded/f_pmsm_foc_sl/MATLAB Function2 ==
  data: ia input; v_alpha output; ib input; ic input; id_ref input; iq_ref input; omega_mech input; theta_mech input; Vdc input; Ld input; Lq input; Rs input; lambda_f input; Tcur input; v_beta output; gg output; dbg output
function [v_alpha, v_beta, gg, dbg] = dpcc_smdo_svpwm(ia, ib, ic, id_ref, iq_ref, ...
                                     omega_mech, theta_mech, Vdc, Ld, Lq, Rs, ...
                                     lambda_f, Tcur)
%#codegen
% Deadbeat predictive current control + your SMDO + SVPWM.
% Drop-in replacement for fcs_smdo_1step: same ports, same SMDO, no cost search.
% lambda_w is unused (deadbeat has no cost function) — kept only for port parity.

omega_r = single(omega_mech);
theta_e = single(mod(theta_mech * 7 - pi/2, 2*pi));
Ts      = single(Tcur);

Vdc = single(Vdc);  Ld = single(Ld);  Lq = single(Lq);  Rs = single(Rs);
lambda_f = single(lambda_f);
id_ref   = single(id_ref);    iq_ref   = single(iq_ref);

% reciprocals (divides ~14 cyc on M4/M7, multiplies ~1) — same idea as yours
inv_Ld  = single(1)/Ld;   inv_Lq  = single(1)/Lq;
inv_Ts  = single(1)/Ts;   inv_Vdc = single(1)/Vdc;
TsLd = Ts*inv_Ld;   TsLq = Ts*inv_Lq;      % Ts/L  (prediction)
LdTs = Ld*inv_Ts;   LqTs = Lq*inv_Ts;      % L/Ts  (deadbeat gain)
INV_SQRT3 = single(0.57735026);            % 1/sqrt(3): linear SVPWM radius / Vdc
SQRT3_2   = single(0.8660254);             % sqrt(3)/2

ct = single(cos(theta_e));  st = single(sin(theta_e));

% ---- Clarke + Park (amplitude-invariant), identical to your FCS ----
i_alpha = (2/3)*(ia - 0.5*ib - 0.5*ic);
i_beta  = (2/3)*(SQRT3_2*(ib - ic));
is_d = single( ct*i_alpha + st*i_beta);
is_q = single(-st*i_alpha + ct*i_beta);
x_k  = single([is_d; is_q]);

% ---- SMDO weights: IDENTICAL to your observer ----
AB = single(0.9);  BB = single(1.2);
K1 = single(6000); K2 = single(6000);
K3 = single(4e6); K4 = single(4e6);

persistent z1 z2 va_prev vb_prev
if isempty(z1)
    z1 = x_k;
    z2 = zeros(2,1,'single');
    va_prev = single(0);   % applied stator voltage (alpha) commanded last step
    vb_prev = single(0);   % applied stator voltage (beta)  commanded last step
end

% ===================== SMDO UPDATE (your observer, verbatim) ================
% v_app: last-commanded stator voltage rotated into dq at the previous angle.
% Replaces (Kcl*s_prev) from the FCS — with SVPWM the applied vector IS the
% continuous alpha-beta reference we stored, so this is exact (no quantization).
th_p = theta_e - omega_r*Ts;
ctp  = single(cos(th_p));  stp = single(sin(th_p));
v_app = single([ctp stp; -stp ctp]) * single([va_prev; vb_prev]);

e = z1 - x_k;
ae = abs(e);  se = sign(e);
sa1 = ae.^AB        .* se;   sb1 = ae.^BB        .* se;
sa2 = ae.^(2*AB-1)  .* se;   sb2 = ae.^(2*BB-1)  .* se;

f_nom = single([(-Rs*x_k(1) + omega_r*Lq*x_k(2))                    *inv_Ld; ...
                (-Rs*x_k(2) - omega_r*Ld*x_k(1) - omega_r*lambda_f) *inv_Lq]);
g_u   = single([v_app(1)*inv_Ld; v_app(2)*inv_Lq]);

z1 = z1 + Ts*(f_nom + g_u + z2 - K1*sa1 - K2*sb1);
z2 = z2 + Ts*(                 - K3*sa2 - K4*sb2);
d_hat = z2;                       % lumped disturbance in di/dt units [A/s]

% ===================== DELAY COMPENSATION: predict i[k+1] ===================
% (analog of your 2-step FCS — deadbeat is delay-sensitive, so keep this on).
% Currently-applied voltage in the CURRENT dq frame:
vdq_now = single([ct st; -st ct]) * single([va_prev; vb_prev]);
id_p = is_d + TsLd*(vdq_now(1) - Rs*is_d + omega_r*Lq*is_q)                     + Ts*d_hat(1);
iq_p = is_q + TsLq*(vdq_now(2) - Rs*is_q - omega_r*Ld*is_d - omega_r*lambda_f)  + Ts*d_hat(2);

% ===================== DEADBEAT: v[k+1] forcing i[k+2] = i_ref ==============
% Same model you invert in the FCS search; solved for voltage instead of picked.
% Disturbance feedforward = -L*d_hat  (d_hat is A/s -> multiply by L for volts).
vd = Rs*id_p - omega_r*Lq*iq_p + LdTs*(id_ref - id_p) - Ld*d_hat(1);
vq = Rs*iq_p + omega_r*Ld*id_p + omega_r*lambda_f + LqTs*(iq_ref - iq_p) - Lq*d_hat(2);

% ===================== HEXAGON CLAMP (inscribed circle = linear SVPWM) ======
Vlim = Vdc*INV_SQRT3;
vmag = single(sqrt(vd*vd + vq*vq));
if vmag > Vlim
    ksc = Vlim/vmag;              % magnitude clamp, angle preserved
    vd = vd*ksc;   vq = vq*ksc;
end

% ===================== ANGLE PREDICTION + inverse Park =====================
% voltage applies over [k+1,k+2]; rotate frame to its midpoint (1.5*Ts).
th  = theta_e + single(1.5)*omega_r*Ts;
cth = single(cos(th));  sth = single(sin(th));
v_alpha = vd*cth - vq*sth;
v_beta  = vd*sth + vq*cth;

va_prev = v_alpha;               % store applied stator voltage for next step
vb_prev = v_beta;

% ===================== SVPWM via min-max injection -> duties ================
va_ph = v_alpha;
vb_ph = -0.5*v_alpha + SQRT3_2*v_beta;
vc_ph = -0.5*v_alpha - SQRT3_2*v_beta;
vmax = max([va_ph, vb_ph, vc_ph]);
vmin = min([va_ph, vb_ph, vc_ph]);
vcom = 0.5*(vmax + vmin);
da = (va_ph - vcom)*inv_Vdc + 0.5;
db = (vb_ph - vcom)*inv_Vdc + 0.5;
dc = (vc_ph - vcom)*inv_Vdc + 0.5;
da = min(max(da,single(0)),single(1));
db = min(max(db,single(0)),single(1));
dc = min(max(dc,single(0)),single(1));

% ===================== OUTPUTS (your port layout) ==========================
% gg now carries DUTY RATIOS + complements (was 0/1 gate logic in the FCS).
% Route gg through a PWM Generator (carrier comparison) -> bridge. See note.
gg = single([da; 1-da; db; 1-db; dc; 1-dc]);

% Commanded fundamental phase voltages (line-to-neutral) for scoping.
%Va = va_ph;   Vb = vb_ph;   Vc = vc_ph;

dbg = single([d_hat(1); d_hat(2); e(1); e(2)]);
end
